simulink model "sm_robot_run_02_aerial_trajectory"  (R2025a)
settings: Solver=ode45  StartTime=0.0  StopTime=2*T_cg-T_stance  MaxStep=0.001  RelTol=1e-3  EnableMultiTasking=on
InitFcn:
  | if (~exist('T_cg') || ~exist('T_stance'))
  |   sm_robot_run_4legs_param_def_load(bdroot)
  | end
undefined symbols (not defined in the file or in its folder): leg_angle0, leg_vel0, T_cg, T_stance
CloseFcn:
  | try,close(h1_sm_robot_run_02_aerial_trajectory),end
  | clear h1_sm_robot_run_02_aerial_trajectory
  | 
  | clear logsout_sm_robot_run_02_aerial_trajectory
Description:
  | Copyright 2012-2025 The MathWorks, Inc.
settings Model: Creator=rhyde  LastModifiedBy=smiller
settings SolverCC: AlgebraicLoopSolver=TrustRegion
settings DataIOCC: SaveFormat=Array  ReturnWorkspaceOutputs=off  SignalLoggingName=logsout_sm_robot_run_02_aerial_trajectory
settings OptimizationCC: ReuseModelBlockBuffer=off  ExpressionDepthLimit=2147483647.0  InitFltsAndDblsToZero=on  LifeSpan=inf
settings DebuggingCC: UnderspecifiedInitializationDetection=Classic  MergeDetectMultiDrivingBlocksExec=none  SolverPrmCheckMsg=warning  FcnCallInpInsideContextMsg=warning  UnconnectedInputMsg=warning  UnconnectedOutputMsg=warning  UnconnectedLineMsg=warning  StateNameClashWarn=warning  PregeneratedLibrarySubsystemCodeDiagnostic=none  SFUnexpectedBacktrackingDiag=warning  SFNoUnconditionalDefaultTransitionDiag=warning  SFExecutionAtInitializationDiag=none  ArithmeticOperatorsInVariantConditions=warning
settings HardwareCC: ProdBitPerPointer=32.0  ProdBitPerSizeT=32.0  ProdBitPerPtrDiffT=32.0  ProdLargestAtomicFloat=None  ProdIntDivRoundTo=Undefined  ProdEndianess=Unspecified  ProdWordSize=32.0  ProdHWDeviceType=32-bit Generic
settings ModelReferenceCC: EnableRefExpFcnMdlSchedulingChecks=on  PropagateSignalLabelsOutOfModel=off
settings SFSimCC: SimUseLocalCustomCode=off  CustomCodeUndefinedFunction=UseInterfaceOnly
settings RTWCC: RTWUseLocalCustomCode=off  GPUComputeCapability=3.5  DLArmComputeVersion=19.05
settings CodeAppCC: StateflowObjectComments=on
settings GRTTargetCC: TargetLangStandard=C89/C90 (ANSI)  CombineOutputUpdateFcns=off  GRTInterface=on
settings ConfigComp: CovMetricSettings=dw  CovSaveCumulativeToWorkspaceVar=on  CovSaveSingleToWorkspaceVar=on  CovExternalEMLEnable=off

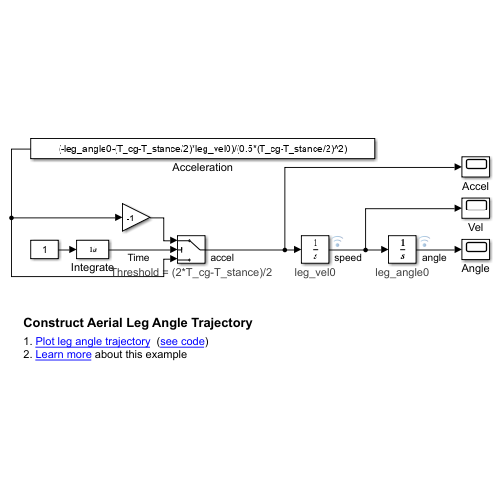
[thumbnail: Simulink's stored preview of the top-level diagram]
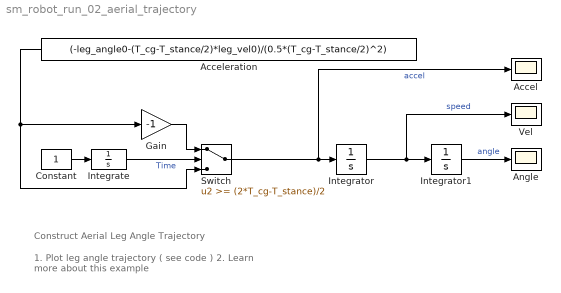
== system sm_robot_run_02_aerial_trajectory ==
  note: Construct Aerial Leg Angle Trajectory
  note: 1. Plot leg angle trajectory ( see code )
      | 2. Learn more about this example
  Accel : Scope
      settings: ActiveDisplayYMinimum=-814.73534  ActiveDisplayYMaximum=814.73534  DataLoggingVariableName=ScopeData2
  Acceleration : Constant  Value=(-leg_angle0-(T_cg-T_stance/2)*leg_vel0)/(0.5*(T_cg-T_stance/2)^2)
  Angle : Scope
      settings: ActiveDisplayYMinimum=-60  ActiveDisplayYMaximum=60  DataLoggingVariableName=aerial_phase_angle
  Constant : Constant
  Gain : Gain  Gain=-1
  Integrate : Integrator
  Integrator : Integrator  InitialCondition=leg_vel0
      settings: AttributesFormatString=%<InitialCondition>
  Integrator1 : Integrator  InitialCondition=leg_angle0
      settings: AttributesFormatString=%<InitialCondition>
  Switch : Switch  Threshold=(2*T_cg-T_stance)/2  SaturateOnIntegerOverflow=off  InputSameDT=off
      settings: AttributesFormatString=Threshold = %<Threshold>
  Vel : Scope
      settings: ActiveDisplayYMinimum=-150  ActiveDisplayYMaximum=200
  wires:
  Integrate/1 -> Switch/2  "Time"
  Acceleration/1 -> Switch/3, Gain/1
  Gain/1 -> Switch/1
  Switch/1 -> Integrator/1, Accel/1  "accel"
  Integrator/1 -> Integrator1/1, Vel/1  "speed"
  Integrator1/1 -> Angle/1  "angle"
  Constant/1 -> Integrate/1
